simulink model "sm_car"  (R2025a)
settings: Solver=ode23t  StartTime=0.0  StopTime=400  MaxStep=0.4  RelTol=1e-3  AbsTol=1e-3  EnableMultiTasking=on
PreLoadFcn:
  | % Due to usability issue in Repeating Sequence block
  | warning('off','Simulink:Masking:Invalid');
  | 
  | % Eliminate unnecessary warnings in inactive variants
  | % Warnings generated only if you click through inactive variant
  | warning('off','MATLAB:nonExistentField');
  | warning('off','Simulink:Parameters:BlkParamUndefined');
PostLoadFcn:
  | set_param([bdroot '/Vehicle'],'popup_trailer','Off')
  | warning('off','sm:sli:setup:compile:LocalSolverNotSupported')
  | %sm_car_config_maneuver(bdroot,'WOT Braking');
  | sm_car_config_vehicle(bdroot,'false');
  | sm_car_config_logging(bdroot);
InitFcn:
  | sm_car_config_camera;
  | Vehicle = sm_car_vehcfg_checkConfig(Vehicle);
  | sm_car_check_tire_model(bdroot);
StartFcn:
  | tic;
StopFcn:
  | Elapsed_Sim_Time = toc;
  | % disp(['Elapsed Sim Time = ' num2str(Elapsed_Sim_Time)]);
undefined symbols (not defined in the file): Axle1D, AxleIn, Camera, Control, Driver, Free, Init, Maneuver, Pedal, RaceFix, RaceSpin, Scene, ShaftL1, ShaftL2, ShaftR1, ShaftR2, Soft, Stiff, Visual, X, xy_data_car_side, Y, Z
libraries: sm_lib x1546, nesl_utility x528, fl_lib x480, SimscapeFluids_lib x61, sdl_lib x49, simulink x29, ee_lib x7, simulink_extras x6, Linkage_Systems x4, Tire_1x2x x4, AntiRollBar_Systems x2, Linkage_Decoupled x2
(part 60 of 79)

== system sm_car/Vehicle/Vehicle/Chassis/SuspA1/Linkage Decoupled/Steer/Rack Driven Shafts/Driver/Human/Torso ==
  ReferenceFrame : sm_lib/Frames and Transforms/Reference Frame
  Solid : sm_lib/Body Elements/File Solid  ExtGeomFileName=Human_torso.STEP  UnitType=Custom  ExtGeomFileUnits=mm  StepReaderType=HEX  ExportConvexHullGeometry=off  InertiaType=CalculateFromGeometry  BasedOnType=Density  Density=rho_human  DensityUnits=kg/m^3  Mass=0  MassUnits=kg  CenterOfMass=[0 0 0]  CenterOfMassUnits=mm  MomentsOfInertia=[1 1 1]  MomentsOfInertiaUnits=kg*mm^2  ProductsOfInertia=[0 0 0]  ProductsOfInertiaUnits=kg*mm^2  GraphicType=FromGeometry  MarkerShape=Sphere  MarkerSize=10  GraphicVisPropType=SimpleVisualProperties  GraphicDiffuseColor=clr_human  GraphicOpacity=opc_human  GraphicSpecularColor=[0.5 0.5 0.5 1.0]  GraphicAmbientColor=[0.15 0.15 0.15 1.0]  GraphicEmissiveColor=[0.0 0.0 0.0 1.0]  GraphicShininess=75  DoExposeReferenceFrame=on  SerializedFrames=<Frames/>
  Transform : sm_lib/Frames and Transforms/Rigid Transform  RotationMethod=ArbitraryAxis  FollAlignAxisA=+X  BaseAlignAxisA=+Y  FollAlignAxisB=+Y  BaseAlignAxisB=+Z  RotationStandardAxis=+Z  RotationAngle=2.0943951023932  RotationAngleUnits=rad  RotationArbitraryAxis=[-0.577350269189626 -0.577350269189626 0.577350269189626]  RotationSequenceAxes=FollowerAxes  RotationSequence=XYX  RotationSequenceAngles=[0 0 0]  RotationSequenceAnglesUnits=deg  RotationMatrix=[1 0 0; 0 1 0; 0 0 1]  Quaternion=[1 0 0 0]  TranslationMethod=Cartesian  TranslationCartesianOffset=[234.912747775434 20.8274805499988 437.3777771]  TranslationCartesianOffsetUnits=mm  TranslationStandardAxis=+Z  TranslationStandardOffset=0  TranslationStandardOffsetUnits=mm  TranslationROffset=0  TranslationROffsetUnits=m  TranslationThetaOffset=0  TranslationThetaOffsetUnits=deg  TranslationZOffset=0  TranslationZOffsetUnits=m
  Transform Neck : sm_lib/Frames and Transforms/Rigid Transform  RotationMethod=StandardAxis  FollAlignAxisA=+X  BaseAlignAxisA=+Y  FollAlignAxisB=+Y  BaseAlignAxisB=+Z  RotationStandardAxis=+X  RotationAngle=90  RotationAngleUnits=deg  RotationArbitraryAxis=[0 0 1]  RotationSequenceAxes=FollowerAxes  RotationSequence=XYX  RotationSequenceAngles=[0 0 0]  RotationSequenceAnglesUnits=deg  RotationMatrix=[1 0 0; 0 1 0; 0 0 1]  Quaternion=[1 0 0 0]  TranslationMethod=None  TranslationCartesianOffset=[0 0 0]  TranslationCartesianOffsetUnits=m  TranslationStandardAxis=+Z  TranslationStandardOffset=0  TranslationStandardOffsetUnits=m  TranslationROffset=0  TranslationROffsetUnits=m  TranslationThetaOffset=0  TranslationThetaOffsetUnits=deg  TranslationZOffset=0  TranslationZOffsetUnits=m
  Transform Nod : sm_lib/Frames and Transforms/Rigid Transform  RotationMethod=StandardAxis  FollAlignAxisA=+X  BaseAlignAxisA=+Y  FollAlignAxisB=+Y  BaseAlignAxisB=+Z  RotationStandardAxis=+Z  RotationAngle=head_incl_angle  RotationAngleUnits=deg  RotationArbitraryAxis=[0 0 1]  RotationSequenceAxes=FollowerAxes  RotationSequence=XYX  RotationSequenceAngles=[0 0 0]  RotationSequenceAnglesUnits=deg  RotationMatrix=[1 0 0; 0 1 0; 0 0 1]  Quaternion=[1 0 0 0]  TranslationMethod=None  TranslationCartesianOffset=[0 0 0]  TranslationCartesianOffsetUnits=m  TranslationStandardAxis=+Z  TranslationStandardOffset=0  TranslationStandardOffsetUnits=m  TranslationROffset=0  TranslationROffsetUnits=m  TranslationThetaOffset=0  TranslationThetaOffsetUnits=deg  TranslationZOffset=0  TranslationZOffsetUnits=m
  Transform ShoulderL : sm_lib/Frames and Transforms/Rigid Transform  RotationMethod=StandardAxis  FollAlignAxisA=+X  BaseAlignAxisA=+Y  FollAlignAxisB=+Y  BaseAlignAxisB=+Z  RotationStandardAxis=+Y  RotationAngle=90  RotationAngleUnits=deg  RotationArbitraryAxis=[0 0 1]  RotationSequenceAxes=FollowerAxes  RotationSequence=XYX  RotationSequenceAngles=[0 0 0]  RotationSequenceAnglesUnits=deg  RotationMatrix=[1 0 0; 0 1 0; 0 0 1]  Quaternion=[1 0 0 0]  TranslationMethod=StandardAxis  TranslationCartesianOffset=[0 0 0]  TranslationCartesianOffsetUnits=m  TranslationStandardAxis=+Z  TranslationStandardOffset=0.05  TranslationStandardOffsetUnits=m  TranslationROffset=0  TranslationROffsetUnits=m  TranslationThetaOffset=0  TranslationThetaOffsetUnits=deg  TranslationZOffset=0  TranslationZOffsetUnits=m
  Transform ShoulderR : sm_lib/Frames and Transforms/Rigid Transform  RotationMethod=StandardAxis  FollAlignAxisA=+X  BaseAlignAxisA=+Y  FollAlignAxisB=+Y  BaseAlignAxisB=+Z  RotationStandardAxis=+Y  RotationAngle=90  RotationAngleUnits=deg  RotationArbitraryAxis=[0 0 1]  RotationSequenceAxes=FollowerAxes  RotationSequence=XYX  RotationSequenceAngles=[0 0 0]  RotationSequenceAnglesUnits=deg  RotationMatrix=[1 0 0; 0 1 0; 0 0 1]  Quaternion=[1 0 0 0]  TranslationMethod=StandardAxis  TranslationCartesianOffset=[0 0 0]  TranslationCartesianOffsetUnits=m  TranslationStandardAxis=+Z  TranslationStandardOffset=0.05  TranslationStandardOffsetUnits=m  TranslationROffset=0  TranslationROffsetUnits=m  TranslationThetaOffset=0  TranslationThetaOffsetUnits=deg  TranslationZOffset=0  TranslationZOffsetUnits=m
  Transform1 : sm_lib/Frames and Transforms/Rigid Transform  RotationMethod=ArbitraryAxis  FollAlignAxisA=+X  BaseAlignAxisA=+Y  FollAlignAxisB=+Y  BaseAlignAxisB=+Z  RotationStandardAxis=+Z  RotationAngle=2.47638432691423  RotationAngleUnits=rad  RotationArbitraryAxis=[-0.663578618400423 -0.663578618400423 -0.345437164189917]  RotationSequenceAxes=FollowerAxes  RotationSequence=XYX  RotationSequenceAngles=[0 0 0]  RotationSequenceAnglesUnits=deg  RotationMatrix=[1 0 0; 0 1 0; 0 0 1]  Quaternion=[1 0 0 0]  TranslationMethod=Cartesian  TranslationCartesianOffset=[3.33060423509468e-15 -64.9684183409698 16.1065362520158]  TranslationCartesianOffsetUnits=mm  TranslationStandardAxis=+Z  TranslationStandardOffset=0  TranslationStandardOffsetUnits=mm  TranslationROffset=0  TranslationROffsetUnits=m  TranslationThetaOffset=0  TranslationThetaOffsetUnits=deg  TranslationZOffset=0  TranslationZOffsetUnits=m
  Transform2 : sm_lib/Frames and Transforms/Rigid Transform  RotationMethod=ArbitraryAxis  FollAlignAxisA=+X  BaseAlignAxisA=+Y  FollAlignAxisB=+Y  BaseAlignAxisB=+Z  RotationStandardAxis=+Z  RotationAngle=2.0943951023932  RotationAngleUnits=rad  RotationArbitraryAxis=[0.577350269189626 0.577350269189626 0.577350269189626]  RotationSequenceAxes=FollowerAxes  RotationSequence=XYX  RotationSequenceAngles=[0 0 0]  RotationSequenceAnglesUnits=deg  RotationMatrix=[1 0 0; 0 1 0; 0 0 1]  Quaternion=[1 0 0 0]  TranslationMethod=Cartesian  TranslationCartesianOffset=[0 20.82747817 499.8600769]  TranslationCartesianOffsetUnits=mm  TranslationStandardAxis=+Z  TranslationStandardOffset=0  TranslationStandardOffsetUnits=mm  TranslationROffset=0  TranslationROffsetUnits=m  TranslationThetaOffset=0  TranslationThetaOffsetUnits=deg  TranslationZOffset=0  TranslationZOffsetUnits=m
  Transform3 : sm_lib/Frames and Transforms/Rigid Transform  RotationMethod=ArbitraryAxis  FollAlignAxisA=+X  BaseAlignAxisA=+Y  FollAlignAxisB=+Y  BaseAlignAxisB=+Z  RotationStandardAxis=+Z  RotationAngle=2.0943951023932  RotationAngleUnits=rad  RotationArbitraryAxis=[0.577350269189626 0.577350269189626 0.577350269189626]  RotationSequenceAxes=FollowerAxes  RotationSequence=XYX  RotationSequenceAngles=[0 0 0]  RotationSequenceAnglesUnits=deg  RotationMatrix=[1 0 0; 0 1 0; 0 0 1]  Quaternion=[1 0 0 0]  TranslationMethod=Cartesian  TranslationCartesianOffset=[-236.437604017244 20.8274805500079 437.377777100002]  TranslationCartesianOffsetUnits=mm  TranslationStandardAxis=+Z  TranslationStandardOffset=0  TranslationStandardOffsetUnits=mm  TranslationROffset=0  TranslationROffsetUnits=m  TranslationThetaOffset=0  TranslationThetaOffsetUnits=deg  TranslationZOffset=0  TranslationZOffsetUnits=m
  Pelvis : PMIOPort  Side=Left
  ArmL : PMIOPort  Port=2  Side=Right
  Head : PMIOPort  Port=3  Side=Right
  ArmR : PMIOPort  Port=4  Side=Right
  connections:
  Transform Nod/RConn1 -- Transform Neck/LConn1
  Transform/LConn1 -- Transform1/LConn1 -- ReferenceFrame/RConn1 -- Solid/RConn1 -- Transform2/LConn1 -- Transform3/LConn1
  Transform ShoulderL/RConn1 -- ArmL/RConn1
  Transform1/RConn1 -- Pelvis/RConn1
  Transform2/RConn1 -- Transform Nod/LConn1
  Transform3/RConn1 -- Transform ShoulderR/LConn1
  Transform ShoulderR/RConn1 -- ArmR/RConn1
  Transform/RConn1 -- Transform ShoulderL/LConn1
  Transform Neck/RConn1 -- Head/RConn1

== system sm_car/Vehicle/Vehicle/Chassis/SuspA1/Linkage Decoupled/Steer/Rack Driven Shafts/Driver/Human/Twist ==
  Revolute Joint : sm_lib/Joints/Revolute Joint  Commented=on  JointMode=Normal  CompositeWrenchDir=FollowerOnBase  CompositeWrenchFrame=BaseFrame  SenseConstraintForce=off  SenseConstraintTorque=off  SenseTotalForce=off  SenseTotalTorque=off  PositionTargetSpecify=off  PositionTargetPriority=High  PositionTargetValue=0  PositionTargetValueUnits=deg  VelocityTargetSpecify=off  VelocityTargetPriority=High  VelocityTargetValue=0  VelocityTargetValueUnits=deg/s  EquilibriumPosition=0  EquilibriumPositionUnits=deg  SpringStiffness=dt_k  SpringStiffnessUnits=N*m/deg  DampingCoefficient=dt_b  DampingCoefficientUnits=N*m/(deg/s)  LowerLimitSpecify=off  LowerLimitBound=-90  LowerLimitBoundUnits=deg  LowerLimitStiffness=1e4  LowerLimitStiffnessUnits=N*m/deg  LowerLimitDamping=10  LowerLimitDampingUnits=N*m/(deg/s)  LowerLimitTransitionRegionWidth=0.1  LowerLimitTransitionRegionWidthUnits=deg  UpperLimitSpecify=off  UpperLimitBound=90  UpperLimitBoundUnits=deg  UpperLimitStiffness=1e4  UpperLimitStiffnessUnits=N*m/deg  UpperLimitDamping=10  UpperLimitDampingUnits=N*m/(deg/s)  UpperLimitTransitionRegionWidth=0.1  UpperLimitTransitionRegionWidthUnits=deg  TorqueActuationMode=NoTorque  MotionActuationMode=ComputedMotion  SensePosition=off  SenseVelocity=off  SenseAcceleration=off  SenseTorqueForce=off  SenseLowerLimitTorqueForce=off  SenseUpperLimitTorqueForce=off
  Transform Axis Location B : sm_lib/Frames and Transforms/Rigid Transform  RotationMethod=None  FollAlignAxisA=+X  BaseAlignAxisA=+Y  FollAlignAxisB=+Y  BaseAlignAxisB=+Z  RotationStandardAxis=+Y  RotationAngle=0  RotationAngleUnits=deg  RotationArbitraryAxis=[0 0 1]  RotationSequenceAxes=FollowerAxes  RotationSequence=XYX  RotationSequenceAngles=[0 0 0]  RotationSequenceAnglesUnits=deg  RotationMatrix=[1 0 0; 0 1 0; 0 0 1]  Quaternion=[1 0 0 0]  TranslationMethod=StandardAxis  TranslationCartesianOffset=[0 0 0]  TranslationCartesianOffsetUnits=m  TranslationStandardAxis=-X  TranslationStandardOffset=0.05  TranslationStandardOffsetUnits=m  TranslationROffset=0  TranslationROffsetUnits=m  TranslationThetaOffset=0  TranslationThetaOffsetUnits=deg  TranslationZOffset=0  TranslationZOffsetUnits=m
  Transform Axis Location F : sm_lib/Frames and Transforms/Rigid Transform  RotationMethod=None  FollAlignAxisA=+X  BaseAlignAxisA=+Y  FollAlignAxisB=+Y  BaseAlignAxisB=+Z  RotationStandardAxis=+Y  RotationAngle=0  RotationAngleUnits=deg  RotationArbitraryAxis=[0 0 1]  RotationSequenceAxes=FollowerAxes  RotationSequence=XYX  RotationSequenceAngles=[0 0 0]  RotationSequenceAnglesUnits=deg  RotationMatrix=[1 0 0; 0 1 0; 0 0 1]  Quaternion=[1 0 0 0]  TranslationMethod=StandardAxis  TranslationCartesianOffset=[0 0 0]  TranslationCartesianOffsetUnits=m  TranslationStandardAxis=-X  TranslationStandardOffset=0.05  TranslationStandardOffsetUnits=m  TranslationROffset=0  TranslationROffsetUnits=m  TranslationThetaOffset=0  TranslationThetaOffsetUnits=deg  TranslationZOffset=0  TranslationZOffsetUnits=m
  Transform Axis Orientation B : sm_lib/Frames and Transforms/Rigid Transform  RotationMethod=StandardAxis  FollAlignAxisA=+X  BaseAlignAxisA=+Y  FollAlignAxisB=+Y  BaseAlignAxisB=+Z  RotationStandardAxis=+Y  RotationAngle=120  RotationAngleUnits=deg  RotationArbitraryAxis=[0 0 1]  RotationSequenceAxes=FollowerAxes  RotationSequence=XYX  RotationSequenceAngles=[0 0 0]  RotationSequenceAnglesUnits=deg  RotationMatrix=[1 0 0; 0 1 0; 0 0 1]  Quaternion=[1 0 0 0]  TranslationMethod=None  TranslationCartesianOffset=[0 0 0]  TranslationCartesianOffsetUnits=m  TranslationStandardAxis=+Z  TranslationStandardOffset=0  TranslationStandardOffsetUnits=m  TranslationROffset=0  TranslationROffsetUnits=m  TranslationThetaOffset=0  TranslationThetaOffsetUnits=deg  TranslationZOffset=0  TranslationZOffsetUnits=m
  Transform Axis Orientation F : sm_lib/Frames and Transforms/Rigid Transform  RotationMethod=StandardAxis  FollAlignAxisA=+X  BaseAlignAxisA=+Y  FollAlignAxisB=+Y  BaseAlignAxisB=+Z  RotationStandardAxis=+Y  RotationAngle=120  RotationAngleUnits=deg  RotationArbitraryAxis=[0 0 1]  RotationSequenceAxes=FollowerAxes  RotationSequence=XYX  RotationSequenceAngles=[0 0 0]  RotationSequenceAnglesUnits=deg  RotationMatrix=[1 0 0; 0 1 0; 0 0 1]  Quaternion=[1 0 0 0]  TranslationMethod=None  TranslationCartesianOffset=[0 0 0]  TranslationCartesianOffsetUnits=m  TranslationStandardAxis=+Z  TranslationStandardOffset=0  TranslationStandardOffsetUnits=m  TranslationROffset=0  TranslationROffsetUnits=m  TranslationThetaOffset=0  TranslationThetaOffsetUnits=deg  TranslationZOffset=0  TranslationZOffsetUnits=m
  Transform Universal B : sm_lib/Frames and Transforms/Rigid Transform  RotationMethod=StandardAxis  FollAlignAxisA=+X  BaseAlignAxisA=+Y  FollAlignAxisB=+Y  BaseAlignAxisB=+Z  RotationStandardAxis=+Y  RotationAngle=90  RotationAngleUnits=deg  RotationArbitraryAxis=[0 0 1]  RotationSequenceAxes=FollowerAxes  RotationSequence=XYX  RotationSequenceAngles=[0 0 0]  RotationSequenceAnglesUnits=deg  RotationMatrix=[1 0 0; 0 1 0; 0 0 1]  Quaternion=[1 0 0 0]  TranslationMethod=None  TranslationCartesianOffset=[0 0 0]  TranslationCartesianOffsetUnits=m  TranslationStandardAxis=+Z  TranslationStandardOffset=0  TranslationStandardOffsetUnits=m  TranslationROffset=0  TranslationROffsetUnits=m  TranslationThetaOffset=0  TranslationThetaOffsetUnits=deg  TranslationZOffset=0  TranslationZOffsetUnits=m
  Transform Universal F : sm_lib/Frames and Transforms/Rigid Transform  RotationMethod=StandardAxis  FollAlignAxisA=+X  BaseAlignAxisA=+Y  FollAlignAxisB=+Y  BaseAlignAxisB=+Z  RotationStandardAxis=+Y  RotationAngle=90  RotationAngleUnits=deg  RotationArbitraryAxis=[0 0 1]  RotationSequenceAxes=FollowerAxes  RotationSequence=XYX  RotationSequenceAngles=[0 0 0]  RotationSequenceAnglesUnits=deg  RotationMatrix=[1 0 0; 0 1 0; 0 0 1]  Quaternion=[1 0 0 0]  TranslationMethod=None  TranslationCartesianOffset=[0 0 0]  TranslationCartesianOffsetUnits=m  TranslationStandardAxis=+Z  TranslationStandardOffset=0  TranslationStandardOffsetUnits=m  TranslationROffset=0  TranslationROffsetUnits=m  TranslationThetaOffset=0  TranslationThetaOffsetUnits=deg  TranslationZOffset=0  TranslationZOffsetUnits=m
  Universal Torso : sm_lib/Joints/Universal Joint  JointMode=Normal  CompositeWrenchDir=FollowerOnBase  CompositeWrenchFrame=BaseFrame  SenseConstraintForce=off  SenseConstraintTorque=off  SenseTotalForce=off  SenseTotalTorque=off  RxPositionTargetSpecify=off  RxPositionTargetPriority=High  RxPositionTargetValue=0  RxPositionTargetValueUnits=deg  RxVelocityTargetSpecify=off  RxVelocityTargetPriority=High  RxVelocityTargetValue=0  RxVelocityTargetValueUnits=deg/s  RxEquilibriumPosition=0  RxEquilibriumPositionUnits=deg  RxSpringStiffness=10  RxSpringStiffnessUnits=N*m/deg  RxDampingCoefficient=1  RxDampingCoefficientUnits=N*m/(deg/s)  RxLowerLimitSpecify=off  RxLowerLimitBound=-90  RxLowerLimitBoundUnits=deg  RxLowerLimitStiffness=1e4  RxLowerLimitStiffnessUnits=N*m/deg  RxLowerLimitDamping=10  RxLowerLimitDampingUnits=N*m/(deg/s)  RxLowerLimitTransitionRegionWidth=0.1  RxLowerLimitTransitionRegionWidthUnits=deg  RxUpperLimitSpecify=off  RxUpperLimitBound=90  RxUpperLimitBoundUnits=deg  RxUpperLimitStiffness=1e4  RxUpperLimitStiffnessUnits=N*m/deg  RxUpperLimitDamping=10  RxUpperLimitDampingUnits=N*m/(deg/s)  RxUpperLimitTransitionRegionWidth=0.1  RxUpperLimitTransitionRegionWidthUnits=deg  RxTorqueActuationMode=NoTorque  RxMotionActuationMode=ComputedMotion  RxSensePosition=off  RxSenseVelocity=off  RxSenseAcceleration=off  RxSenseTorqueForce=off  RxSenseLowerLimitTorqueForce=off  RxSenseUpperLimitTorqueForce=off  RyPositionTargetSpecify=off  RyPositionTargetPriority=High  RyPositionTargetValue=0  RyPositionTargetValueUnits=deg  RyVelocityTargetSpecify=off  RyVelocityTargetPriority=High  RyVelocityTargetValue=0  RyVelocityTargetValueUnits=deg/s  RyEquilibriumPosition=0  RyEquilibriumPositionUnits=deg  RySpringStiffness=10  RySpringStiffnessUnits=N*m/deg  RyDampingCoefficient=1  RyDampingCoefficientUnits=N*m/(deg/s)  RyLowerLimitSpecify=off  RyLowerLimitBound=-90  RyLowerLimitBoundUnits=deg  RyLowerLimitStiffness=1e4  RyLowerLimitStiffnessUnits=N*m/deg  RyLowerLimitDamping=10  RyLowerLimitDampingUnits=N*m/(deg/s)  RyLowerLimitTransitionRegionWidth=0.1  RyLowerLimitTransitionRegionWidthUnits=deg  RyUpperLimitSpecify=off  RyUpperLimitBound=90  RyUpperLimitBoundUnits=deg  RyUpperLimitStiffness=1e4  RyUpperLimitStiffnessUnits=N*m/deg  RyUpperLimitDamping=10  RyUpperLimitDampingUnits=N*m/(deg/s)  RyUpperLimitTransitionRegionWidth=0.1  RyUpperLimitTransitionRegionWidthUnits=deg  RyTorqueActuationMode=NoTorque  RyMotionActuationMode=ComputedMotion  RySensePosition=off  RySenseVelocity=off  RySenseAcceleration=off  RySenseTorqueForce=off  RySenseLowerLimitTorqueForce=off  RySenseUpperLimitTorqueForce=off
  T : PMIOPort  Side=Right
  B : PMIOPort  Port=2  Side=Left
  connections:
  Universal Torso/RConn1 -- Transform Universal F/RConn1
  Universal Torso/LConn1 -- Transform Universal B/RConn1
  Transform Axis Location F/RConn1 -- Transform Universal F/LConn1
  Transform Axis Orientation F/LConn1 -- T/RConn1
  Transform Axis Location B/RConn1 -- Transform Universal B/LConn1
  Transform Axis Orientation F/RConn1 -- Transform Axis Location F/LConn1
  B/RConn1 -- Transform Axis Orientation B/LConn1
  Transform Axis Orientation B/RConn1 -- Transform Axis Location B/LConn1

== system sm_car/Vehicle/Vehicle/Chassis/SuspA1/Linkage Decoupled/Steer/Rack Driven Shafts/Driver/None/Body Sensor Empty ==
  Constant{,1..14} (15 alike) : Constant  Value=0
  Reference Frame : sm_lib/Frames and Transforms/Reference Frame
  Signal Specification : SignalSpecification  Unit=rad
  Signal Specification1 : SignalSpecification  Unit=rad
  Signal Specification2 : SignalSpecification  Unit=rad
  Signal Specification3 : SignalSpecification  Unit=rad/s
  Signal Specification4 : SignalSpecification  Unit=rad/s
  Signal Specification5 : SignalSpecification  Unit=rad/s
  B : PMIOPort  Side=Left
  Bus Element Out : Outport  VectorParamsAs1DForOutWhenUnconnected=off  PortName=Body  Element=x
  Bus Element Out1 : Outport  VectorParamsAs1DForOutWhenUnconnected=off  PortName=Body  Element=y
  Bus Element Out2 : Outport  VectorParamsAs1DForOutWhenUnconnected=off  PortName=Body  Element=z
  Bus Element Out3 : Outport  VectorParamsAs1DForOutWhenUnconnected=off  PortName=Body  Element=vx
  Bus Element Out4 : Outport  VectorParamsAs1DForOutWhenUnconnected=off  PortName=Body  Element=vy
  Bus Element Out5 : Outport  VectorParamsAs1DForOutWhenUnconnected=off  PortName=Body  Element=vz
  Bus Element Out6 : Outport  VectorParamsAs1DForOutWhenUnconnected=off  PortName=Body  Element=gx
  Bus Element Out7 : Outport  VectorParamsAs1DForOutWhenUnconnected=off  PortName=Body  Element=gy
  Bus Element Out8 : Outport  VectorParamsAs1DForOutWhenUnconnected=off  PortName=Body  Element=gz
  Bus Element Out9 : Outport  VectorParamsAs1DForOutWhenUnconnected=off  PortName=Body  Element=nRoll
  Bus Element Out10 : Outport  VectorParamsAs1DForOutWhenUnconnected=off  PortName=Body  Element=nPitch
  Bus Element Out11 : Outport  VectorParamsAs1DForOutWhenUnconnected=off  PortName=Body  Element=nYaw
  Bus Element Out12 : Outport  VectorParamsAs1DForOutWhenUnconnected=off  PortName=Body  Element=aRoll
  Bus Element Out13 : Outport  VectorParamsAs1DForOutWhenUnconnected=off  PortName=Body  Element=aPitch
  Bus Element Out14 : Outport  VectorParamsAs1DForOutWhenUnconnected=off  PortName=Body  Element=aYaw
  wires:
  Constant2/1 -> Signal Specification/1
  Constant3/1 -> Signal Specification1/1
  Constant5/1 -> Signal Specification4/1
  Constant4/1 -> Signal Specification3/1
  Constant1/1 -> Signal Specification5/1
  Constant/1 -> Signal Specification2/1
  Signal Specification5/1 -> Bus Element Out11/1
  Signal Specification4/1 -> Bus Element Out10/1
  Signal Specification3/1 -> Bus Element Out9/1
  Signal Specification2/1 -> Bus Element Out14/1
  Signal Specification1/1 -> Bus Element Out13/1
  Signal Specification/1 -> Bus Element Out12/1
  Constant9/1 -> Bus Element Out3/1
  Constant6/1 -> Bus Element Out/1
  Constant8/1 -> Bus Element Out2/1
  Constant10/1 -> Bus Element Out4/1
  Constant13/1 -> Bus Element Out7/1
  Constant7/1 -> Bus Element Out1/1
  Constant12/1 -> Bus Element Out6/1
  Constant11/1 -> Bus Element Out5/1
  Constant14/1 -> Bus Element Out8/1
  connections:
  B/RConn1 -- Reference Frame/RConn1

== system sm_car/Vehicle/Vehicle/Chassis/SuspA1/Linkage Decoupled/Steer/Rack Driven Shafts/Wheel/FSAE/Transform Steer Axis ==
  Rigid Transform1 : sm_lib/Frames and Transforms/Rigid Transform  RotationMethod=None  FollAlignAxisA=+X  BaseAlignAxisA=+Y  FollAlignAxisB=+Y  BaseAlignAxisB=+Z  RotationStandardAxis=+Z  RotationAngle=0.0  RotationAngleUnits=deg  RotationArbitraryAxis=[0 0 1]  RotationSequenceAxes=FollowerAxes  RotationSequence=XYX  RotationSequenceAngles=[0 0 0]  RotationSequenceAnglesUnits=deg  RotationMatrix=[1 0 0; 0 1 0; 0 0 1]  Quaternion=[1 0 0 0]  TranslationMethod=Cartesian  TranslationCartesianOffset=[0 -0.4664 -0.3791]  TranslationCartesianOffsetUnits=m  TranslationStandardAxis=+Z  TranslationStandardOffset=0  TranslationStandardOffsetUnits=m  TranslationROffset=0  TranslationROffsetUnits=m  TranslationThetaOffset=0  TranslationThetaOffsetUnits=deg  TranslationZOffset=0  TranslationZOffsetUnits=m
  Rigid Transform2 : sm_lib/Frames and Transforms/Rigid Transform  RotationMethod=RotationMatrix  FollAlignAxisA=+X  BaseAlignAxisA=+Y  FollAlignAxisB=+Y  BaseAlignAxisB=+Z  RotationStandardAxis=+Z  RotationAngle=0.0  RotationAngleUnits=deg  RotationArbitraryAxis=[0 0 1]  RotationSequenceAxes=FollowerAxes  RotationSequence=XYX  RotationSequenceAngles=[0 0 0]  RotationSequenceAnglesUnits=deg  RotationMatrix=[0.5 0.866 -6.661e-16; -0.8602 0.4967 0.1153; 0.09988 -0.05766 0.9933]  Quaternion=[1 0 0 0]  TranslationMethod=None  TranslationCartesianOffset=[0 0 0]  TranslationCartesianOffsetUnits=m  TranslationStandardAxis=+Z  TranslationStandardOffset=0  TranslationStandardOffsetUnits=m  TranslationROffset=0  TranslationROffsetUnits=m  TranslationThetaOffset=0  TranslationThetaOffsetUnits=deg  TranslationZOffset=0  TranslationZOffsetUnits=m
  Rigid Transform4 : sm_lib/Frames and Transforms/Rigid Transform  RotationMethod=StandardAxis  FollAlignAxisA=+X  BaseAlignAxisA=+Y  FollAlignAxisB=+Y  BaseAlignAxisB=+Z  RotationStandardAxis=+Z  RotationAngle=150  RotationAngleUnits=deg  RotationArbitraryAxis=[0 0 1]  RotationSequenceAxes=FollowerAxes  RotationSequence=XYX  RotationSequenceAngles=[0 0 0]  RotationSequenceAnglesUnits=deg  RotationMatrix=[1 0 0; 0 1 0; 0 0 1]  Quaternion=[1 0 0 0]  TranslationMethod=StandardAxis  TranslationCartesianOffset=[0 0 0]  TranslationCartesianOffsetUnits=m  TranslationStandardAxis=+Z  TranslationStandardOffset=0.09  TranslationStandardOffsetUnits=m  TranslationROffset=0  TranslationROffsetUnits=m  TranslationThetaOffset=0  TranslationThetaOffsetUnits=deg  TranslationZOffset=0  TranslationZOffsetUnits=m
  F : PMIOPort  Side=Left
  B : PMIOPort  Port=2  Side=Right
  connections:
  B/RConn1 -- Rigid Transform1/RConn1
  Rigid Transform1/LConn1 -- Rigid Transform2/LConn1
  F/RConn1 -- Rigid Transform4/RConn1
  Rigid Transform2/RConn1 -- Rigid Transform4/LConn1

== system sm_car/Vehicle/Vehicle/Chassis/SuspA1/Linkage Decoupled/Steer/Rack Driven Shafts/Wheel/Sedan/Steering ==
  Steering Wheel : sm_lib/Body Elements/File Solid  ExtGeomFileName=Sedan_Hamba_Steering_Wheel.stl  UnitType=Custom  ExtGeomFileUnits=m  StepReaderType=HEX  ExportConvexHullGeometry=off  InertiaType=CalculateFromGeometry  BasedOnType=Density  Density=1000  DensityUnits=kg/m^3  Mass=0  MassUnits=kg  CenterOfMass=[0 0 0]  CenterOfMassUnits=m  MomentsOfInertia=[1 1 1]  MomentsOfInertiaUnits=kg*m^2  ProductsOfInertia=[0 0 0]  ProductsOfInertiaUnits=kg*m^2  GraphicType=FromGeometry  MarkerShape=Sphere  MarkerSize=10  GraphicVisPropType=SimpleVisualProperties  GraphicDiffuseColor=[0.4 0.4 0.4]  GraphicOpacity=1.0  GraphicSpecularColor=[0.5 0.5 0.5 1.0]  GraphicAmbientColor=[0.15 0.15 0.15 1.0]  GraphicEmissiveColor=[0.0 0.0 0.0 1.0]  GraphicShininess=75  DoExposeReferenceFrame=on  SerializedFrames=<Frames/>
  Transform Bot Ctr : sm_lib/Frames and Transforms/Rigid Transform  RotationMethod=None  FollAlignAxisA=+X  BaseAlignAxisA=+Y  FollAlignAxisB=+Y  BaseAlignAxisB=+Z  RotationStandardAxis=+Z  RotationAngle=0.0  RotationAngleUnits=deg  RotationArbitraryAxis=[0 0 1]  RotationSequenceAxes=FollowerAxes  RotationSequence=XYX  RotationSequenceAngles=[0 0 0]  RotationSequenceAnglesUnits=deg  RotationMatrix=[1 0 0; 0 1 0; 0 0 1]  Quaternion=[1 0 0 0]  TranslationMethod=Cartesian  TranslationCartesianOffset="[-0.020653016865253  -0.076110564172268   0.210841685533524]"  TranslationCartesianOffsetUnits=m  TranslationStandardAxis=+Z  TranslationStandardOffset=0  TranslationStandardOffsetUnits=m  TranslationROffset=0  TranslationROffsetUnits=m  TranslationThetaOffset=0  TranslationThetaOffsetUnits=deg  TranslationZOffset=0  TranslationZOffsetUnits=m
  Transform Location : sm_lib/Frames and Transforms/Rigid Transform  RotationMethod=None  FollAlignAxisA=+X  BaseAlignAxisA=+Y  FollAlignAxisB=+Y  BaseAlignAxisB=+Z  RotationStandardAxis=+Z  RotationAngle=0.0  RotationAngleUnits=deg  RotationArbitraryAxis=[0 0 1]  RotationSequenceAxes=FollowerAxes  RotationSequence=XYX  RotationSequenceAngles=[0 0 0]  RotationSequenceAnglesUnits=deg  RotationMatrix=[1 0 0; 0 1 0; 0 0 1]  Quaternion=[1 0 0 0]  TranslationMethod=Cartesian  TranslationCartesianOffset=[0.5868 -0.3915 -0.838]  TranslationCartesianOffsetUnits=m  TranslationStandardAxis=+Z  TranslationStandardOffset=0  TranslationStandardOffsetUnits=m  TranslationROffset=0  TranslationROffsetUnits=m  TranslationThetaOffset=0  TranslationThetaOffsetUnits=deg  TranslationZOffset=0  TranslationZOffsetUnits=m
  Transform Orientation : sm_lib/Frames and Transforms/Rigid Transform  RotationMethod=RotationSequence  FollAlignAxisA=+X  BaseAlignAxisA=+Y  FollAlignAxisB=+Y  BaseAlignAxisB=+Z  RotationStandardAxis=+Z  RotationAngle=0.0  RotationAngleUnits=deg  RotationArbitraryAxis=[0 0 1]  RotationSequenceAxes=FollowerAxes  RotationSequence=ZYX  RotationSequenceAngles=[-90 -90 0]  RotationSequenceAnglesUnits=deg  RotationMatrix=[1 0 0; 0 1 0; 0 0 1]  Quaternion=[1 0 0 0]  TranslationMethod=None  TranslationCartesianOffset=[0 0 0]  TranslationCartesianOffsetUnits=m  TranslationStandardAxis=+Z  TranslationStandardOffset=0  TranslationStandardOffsetUnits=m  TranslationROffset=0  TranslationROffsetUnits=m  TranslationThetaOffset=0  TranslationThetaOffsetUnits=deg  TranslationZOffset=0  TranslationZOffsetUnits=m
  Transform Top Ctr : sm_lib/Frames and Transforms/Rigid Transform  RotationMethod=None  FollAlignAxisA=+X  BaseAlignAxisA=+Y  FollAlignAxisB=+Y  BaseAlignAxisB=+Z  RotationStandardAxis=+Z  RotationAngle=0.0  RotationAngleUnits=deg  RotationArbitraryAxis=[0 0 1]  RotationSequenceAxes=FollowerAxes  RotationSequence=XYX  RotationSequenceAngles=[0 0 0]  RotationSequenceAnglesUnits=deg  RotationMatrix=[1 0 0; 0 1 0; 0 0 1]  Quaternion=[1 0 0 0]  TranslationMethod=Cartesian  TranslationCartesianOffset="[0.124706447124481   0.318579733371735   0.210841685533524]"  TranslationCartesianOffsetUnits=m  TranslationStandardAxis=+Z  TranslationStandardOffset=0  TranslationStandardOffsetUnits=m  TranslationROffset=0  TranslationROffsetUnits=m  TranslationThetaOffset=0  TranslationThetaOffsetUnits=deg  TranslationZOffset=0  TranslationZOffsetUnits=m
  R : PMIOPort  Side=Right
  BotCtr : PMIOPort  Port=2  Side=Left
  TopCtr : PMIOPort  Port=3  Side=Left
  connections:
  Transform Bot Ctr/LConn1 -- Transform Orientation/LConn1 -- R/RConn1 -- Transform Top Ctr/LConn1
  Transform Location/RConn1 -- Steering Wheel/RConn1
  Transform Orientation/RConn1 -- Transform Location/LConn1
  Transform Bot Ctr/RConn1 -- BotCtr/RConn1
  TopCtr/RConn1 -- Transform Top Ctr/RConn1

== system sm_car/Vehicle/Vehicle/Chassis/SuspA1/Linkage Decoupled/Steer/Rack Static Shafts/Driver/Human/Arm L ==
  Arm Lower L : Subsystem
  Arm Upper L : Subsystem
  Hand L : Subsystem
  Revolute ElbowL : sm_lib/Joints/Revolute Joint  JointMode=Normal  CompositeWrenchDir=FollowerOnBase  CompositeWrenchFrame=BaseFrame  SenseConstraintForce=off  SenseConstraintTorque=off  SenseTotalForce=off  SenseTotalTorque=off  PositionTargetSpecify=on  PositionTargetPriority=Low  PositionTargetValue=50  PositionTargetValueUnits=deg  VelocityTargetSpecify=off  VelocityTargetPriority=High  VelocityTargetValue=0  VelocityTargetValueUnits=deg/s  EquilibriumPosition=0  EquilibriumPositionUnits=deg  SpringStiffness=0  SpringStiffnessUnits=N*m/deg  DampingCoefficient=0  DampingCoefficientUnits=N*m/(deg/s)  LowerLimitSpecify=off  LowerLimitBound=-90  LowerLimitBoundUnits=deg  LowerLimitStiffness=1e4  LowerLimitStiffnessUnits=N*m/deg  LowerLimitDamping=10  LowerLimitDampingUnits=N*m/(deg/s)  LowerLimitTransitionRegionWidth=0.1  LowerLimitTransitionRegionWidthUnits=deg  UpperLimitSpecify=off  UpperLimitBound=90  UpperLimitBoundUnits=deg  UpperLimitStiffness=1e4  UpperLimitStiffnessUnits=N*m/deg  UpperLimitDamping=10  UpperLimitDampingUnits=N*m/(deg/s)  UpperLimitTransitionRegionWidth=0.1  UpperLimitTransitionRegionWidthUnits=deg  TorqueActuationMode=NoTorque  MotionActuationMode=ComputedMotion  SensePosition=off  SenseVelocity=off  SenseAcceleration=off  SenseTorqueForce=off  SenseLowerLimitTorqueForce=off  SenseUpperLimitTorqueForce=off
  Spherical ShoulderL : sm_lib/Joints/Spherical Joint  JointMode=Normal  CompositeWrenchDir=FollowerOnBase  CompositeWrenchFrame=BaseFrame  SenseConstraintForce=off  SenseConstraintTorque=off  SenseTotalForce=off  SenseTotalTorque=off  PositionTargetSpecify=off  PositionTargetPriority=High  PositionTargetRotationMethod=None  PositionTargetFollAlignAxisA=+X  PositionTargetBaseAlignAxisA=+Y  PositionTargetFollAlignAxisB=+Y  PositionTargetBaseAlignAxisB=+Z  PositionTargetRotationStandardAxis=+Z  PositionTargetRotationAngle=0.0  PositionTargetRotationAngleUnits=deg  PositionTargetRotationArbitraryAxis=[0 0 1]  PositionTargetRotationSequenceAxes=FollowerAxes  PositionTargetRotationSequence=XYX  PositionTargetRotationSequenceAngles=[0 0 0]  PositionTargetRotationSequenceAnglesUnits=deg  PositionTargetRotationMatrix=[1 0 0; 0 1 0; 0 0 1]  PositionTargetQuaternion=[1 0 0 0]  VelocityTargetSpecify=off  VelocityTargetPriority=High  VelocityTargetValue=[0 0 0]  VelocityTargetValueUnits=deg/s  VelocityTargetInFollowerFrame=on  EqPosRotationMethod=None  EqPosFollAlignAxisA=+X  EqPosBaseAlignAxisA=+Y  EqPosFollAlignAxisB=+Y  EqPosBaseAlignAxisB=+Z  EqPosRotationStandardAxis=+Z  EqPosRotationAngle=0.0  EqPosRotationAngleUnits=deg  EqPosRotationArbitraryAxis=[0 0 1]  EqPosRotationSequenceAxes=FollowerAxes  EqPosRotationSequence=XYX  EqPosRotationSequenceAngles=[0 0 0]  EqPosRotationSequenceAnglesUnits=deg  EqPosRotationMatrix=[1 0 0; 0 1 0; 0 0 1]  EqPosQuaternion=[1 0 0 0]  SpringStiffness=0  SpringStiffnessUnits=N*m/deg  DampingCoefficient=0  DampingCoefficientUnits=N*m/(deg/s)  LowerLimitSpecify=off  LowerLimitBound=15  LowerLimitBoundUnits=deg  LowerLimitStiffness=1e4  LowerLimitStiffnessUnits=N*m/deg  LowerLimitDamping=10  LowerLimitDampingUnits=N*m/(deg/s)  LowerLimitTransitionRegionWidth=0.1  LowerLimitTransitionRegionWidthUnits=deg  UpperLimitSpecify=off  UpperLimitBound=45  UpperLimitBoundUnits=deg  UpperLimitStiffness=1e4  UpperLimitStiffnessUnits=N*m/deg  UpperLimitDamping=10  UpperLimitDampingUnits=N*m/(deg/s)  UpperLimitTransitionRegionWidth=0.1  UpperLimitTransitionRegionWidthUnits=deg  TorqueActuationMode=NoTorque  ActuateTorqueX=off  ActuateTorqueY=off  ActuateTorqueZ=off  ActuateTorque=off  ActuationFrame=BaseFrame  SensePosition=off  SenseVelocityX=off  SenseVelocityY=off  SenseVelocityZ=off  SenseVelocity=off  SenseAccelerationX=off  SenseAccelerationY=off  SenseAccelerationZ=off  SenseAcceleration=off  SenseLowerLimitTorqueMag=off  SenseUpperLimitTorqueMag=off  SensingFrame=BaseFrame
  Universal WristL : sm_lib/Joints/Universal Joint  JointMode=Normal  CompositeWrenchDir=FollowerOnBase  CompositeWrenchFrame=BaseFrame  SenseConstraintForce=off  SenseConstraintTorque=off  SenseTotalForce=off  SenseTotalTorque=off  RxPositionTargetSpecify=off  RxPositionTargetPriority=High  RxPositionTargetValue=0  RxPositionTargetValueUnits=deg  RxVelocityTargetSpecify=off  RxVelocityTargetPriority=High  RxVelocityTargetValue=0  RxVelocityTargetValueUnits=deg/s  RxEquilibriumPosition=0  RxEquilibriumPositionUnits=deg  RxSpringStiffness=0  RxSpringStiffnessUnits=N*m/deg  RxDampingCoefficient=0  RxDampingCoefficientUnits=N*m/(deg/s)  RxLowerLimitSpecify=off  RxLowerLimitBound=-90  RxLowerLimitBoundUnits=deg  RxLowerLimitStiffness=1e4  RxLowerLimitStiffnessUnits=N*m/deg  RxLowerLimitDamping=10  RxLowerLimitDampingUnits=N*m/(deg/s)  RxLowerLimitTransitionRegionWidth=0.1  RxLowerLimitTransitionRegionWidthUnits=deg  RxUpperLimitSpecify=off  RxUpperLimitBound=90  RxUpperLimitBoundUnits=deg  RxUpperLimitStiffness=1e4  RxUpperLimitStiffnessUnits=N*m/deg  RxUpperLimitDamping=10  RxUpperLimitDampingUnits=N*m/(deg/s)  RxUpperLimitTransitionRegionWidth=0.1  RxUpperLimitTransitionRegionWidthUnits=deg  RxTorqueActuationMode=NoTorque  RxMotionActuationMode=ComputedMotion  RxSensePosition=off  RxSenseVelocity=off  RxSenseAcceleration=off  RxSenseTorqueForce=off  RxSenseLowerLimitTorqueForce=off  RxSenseUpperLimitTorqueForce=off  RyPositionTargetSpecify=off  RyPositionTargetPriority=High  RyPositionTargetValue=0  RyPositionTargetValueUnits=deg  RyVelocityTargetSpecify=off  RyVelocityTargetPriority=High  RyVelocityTargetValue=0  RyVelocityTargetValueUnits=deg/s  RyEquilibriumPosition=0  RyEquilibriumPositionUnits=deg  RySpringStiffness=0  RySpringStiffnessUnits=N*m/deg  RyDampingCoefficient=0  RyDampingCoefficientUnits=N*m/(deg/s)  RyLowerLimitSpecify=off  RyLowerLimitBound=-90  RyLowerLimitBoundUnits=deg  RyLowerLimitStiffness=1e4  RyLowerLimitStiffnessUnits=N*m/deg  RyLowerLimitDamping=10  RyLowerLimitDampingUnits=N*m/(deg/s)  RyLowerLimitTransitionRegionWidth=0.1  RyLowerLimitTransitionRegionWidthUnits=deg  RyUpperLimitSpecify=off  RyUpperLimitBound=90  RyUpperLimitBoundUnits=deg  RyUpperLimitStiffness=1e4  RyUpperLimitStiffnessUnits=N*m/deg  RyUpperLimitDamping=10  RyUpperLimitDampingUnits=N*m/(deg/s)  RyUpperLimitTransitionRegionWidth=0.1  RyUpperLimitTransitionRegionWidthUnits=deg  RyTorqueActuationMode=NoTorque  RyMotionActuationMode=ComputedMotion  RySensePosition=off  RySenseVelocity=off  RySenseAcceleration=off  RySenseTorqueForce=off  RySenseLowerLimitTorqueForce=off  RySenseUpperLimitTorqueForce=off
  Sh : PMIOPort  Side=Left
  Grip : PMIOPort  Port=2  Side=Right
  connections:
  Revolute ElbowL/LConn1 -- Arm Upper L/RConn1
  Spherical ShoulderL/RConn1 -- Arm Upper L/LConn1
  Universal WristL/RConn1 -- Hand L/LConn1
  Hand L/RConn1 -- Grip/RConn1
  Arm Lower L/LConn1 -- Revolute ElbowL/RConn1
  Arm Lower L/RConn1 -- Universal WristL/LConn1
  Spherical ShoulderL/LConn1 -- Sh/RConn1

== system sm_car/Vehicle/Vehicle/Chassis/SuspA1/Linkage Decoupled/Steer/Rack Static Shafts/Driver/Human/Arm R ==
  Arm Lower R : Subsystem
  Arm Upper R : Subsystem
  Hand R : Subsystem
  Revolute ElbowR : sm_lib/Joints/Revolute Joint  JointMode=Normal  CompositeWrenchDir=FollowerOnBase  CompositeWrenchFrame=BaseFrame  SenseConstraintForce=off  SenseConstraintTorque=off  SenseTotalForce=off  SenseTotalTorque=off  PositionTargetSpecify=on  PositionTargetPriority=Low  PositionTargetValue=50  PositionTargetValueUnits=deg  VelocityTargetSpecify=off  VelocityTargetPriority=High  VelocityTargetValue=0  VelocityTargetValueUnits=deg/s  EquilibriumPosition=0  EquilibriumPositionUnits=deg  SpringStiffness=0  SpringStiffnessUnits=N*m/deg  DampingCoefficient=0  DampingCoefficientUnits=N*m/(deg/s)  LowerLimitSpecify=off  LowerLimitBound=-90  LowerLimitBoundUnits=deg  LowerLimitStiffness=1e4  LowerLimitStiffnessUnits=N*m/deg  LowerLimitDamping=10  LowerLimitDampingUnits=N*m/(deg/s)  LowerLimitTransitionRegionWidth=0.1  LowerLimitTransitionRegionWidthUnits=deg  UpperLimitSpecify=off  UpperLimitBound=90  UpperLimitBoundUnits=deg  UpperLimitStiffness=1e4  UpperLimitStiffnessUnits=N*m/deg  UpperLimitDamping=10  UpperLimitDampingUnits=N*m/(deg/s)  UpperLimitTransitionRegionWidth=0.1  UpperLimitTransitionRegionWidthUnits=deg  TorqueActuationMode=NoTorque  MotionActuationMode=ComputedMotion  SensePosition=off  SenseVelocity=off  SenseAcceleration=off  SenseTorqueForce=off  SenseLowerLimitTorqueForce=off  SenseUpperLimitTorqueForce=off
  Spherical ShoulderR : sm_lib/Joints/Spherical Joint  JointMode=Normal  CompositeWrenchDir=FollowerOnBase  CompositeWrenchFrame=BaseFrame  SenseConstraintForce=off  SenseConstraintTorque=off  SenseTotalForce=off  SenseTotalTorque=off  PositionTargetSpecify=off  PositionTargetPriority=High  PositionTargetRotationMethod=None  PositionTargetFollAlignAxisA=+X  PositionTargetBaseAlignAxisA=+Y  PositionTargetFollAlignAxisB=+Y  PositionTargetBaseAlignAxisB=+Z  PositionTargetRotationStandardAxis=+Z  PositionTargetRotationAngle=0.0  PositionTargetRotationAngleUnits=deg  PositionTargetRotationArbitraryAxis=[0 0 1]  PositionTargetRotationSequenceAxes=FollowerAxes  PositionTargetRotationSequence=XYX  PositionTargetRotationSequenceAngles=[0 0 0]  PositionTargetRotationSequenceAnglesUnits=deg  PositionTargetRotationMatrix=[1 0 0; 0 1 0; 0 0 1]  PositionTargetQuaternion=[1 0 0 0]  VelocityTargetSpecify=off  VelocityTargetPriority=High  VelocityTargetValue=[0 0 0]  VelocityTargetValueUnits=deg/s  VelocityTargetInFollowerFrame=on  EqPosRotationMethod=None  EqPosFollAlignAxisA=+X  EqPosBaseAlignAxisA=+Y  EqPosFollAlignAxisB=+Y  EqPosBaseAlignAxisB=+Z  EqPosRotationStandardAxis=+Z  EqPosRotationAngle=0.0  EqPosRotationAngleUnits=deg  EqPosRotationArbitraryAxis=[0 0 1]  EqPosRotationSequenceAxes=FollowerAxes  EqPosRotationSequence=XYX  EqPosRotationSequenceAngles=[0 0 0]  EqPosRotationSequenceAnglesUnits=deg  EqPosRotationMatrix=[1 0 0; 0 1 0; 0 0 1]  EqPosQuaternion=[1 0 0 0]  SpringStiffness=0  SpringStiffnessUnits=N*m/deg  DampingCoefficient=0  DampingCoefficientUnits=N*m/(deg/s)  LowerLimitSpecify=off  LowerLimitBound=15  LowerLimitBoundUnits=deg  LowerLimitStiffness=1e4  LowerLimitStiffnessUnits=N*m/deg  LowerLimitDamping=10  LowerLimitDampingUnits=N*m/(deg/s)  LowerLimitTransitionRegionWidth=0.1  LowerLimitTransitionRegionWidthUnits=deg  UpperLimitSpecify=off  UpperLimitBound=45  UpperLimitBoundUnits=deg  UpperLimitStiffness=1e4  UpperLimitStiffnessUnits=N*m/deg  UpperLimitDamping=10  UpperLimitDampingUnits=N*m/(deg/s)  UpperLimitTransitionRegionWidth=0.1  UpperLimitTransitionRegionWidthUnits=deg  TorqueActuationMode=NoTorque  ActuateTorqueX=off  ActuateTorqueY=off  ActuateTorqueZ=off  ActuateTorque=off  ActuationFrame=BaseFrame  SensePosition=off  SenseVelocityX=off  SenseVelocityY=off  SenseVelocityZ=off  SenseVelocity=off  SenseAccelerationX=off  SenseAccelerationY=off  SenseAccelerationZ=off  SenseAcceleration=off  SenseLowerLimitTorqueMag=off  SenseUpperLimitTorqueMag=off  SensingFrame=BaseFrame
  Universal WristR : sm_lib/Joints/Universal Joint  JointMode=Normal  CompositeWrenchDir=FollowerOnBase  CompositeWrenchFrame=BaseFrame  SenseConstraintForce=off  SenseConstraintTorque=off  SenseTotalForce=off  SenseTotalTorque=off  RxPositionTargetSpecify=off  RxPositionTargetPriority=High  RxPositionTargetValue=0  RxPositionTargetValueUnits=deg  RxVelocityTargetSpecify=off  RxVelocityTargetPriority=High  RxVelocityTargetValue=0  RxVelocityTargetValueUnits=deg/s  RxEquilibriumPosition=0  RxEquilibriumPositionUnits=deg  RxSpringStiffness=0  RxSpringStiffnessUnits=N*m/deg  RxDampingCoefficient=0  RxDampingCoefficientUnits=N*m/(deg/s)  RxLowerLimitSpecify=off  RxLowerLimitBound=-90  RxLowerLimitBoundUnits=deg  RxLowerLimitStiffness=1e4  RxLowerLimitStiffnessUnits=N*m/deg  RxLowerLimitDamping=10  RxLowerLimitDampingUnits=N*m/(deg/s)  RxLowerLimitTransitionRegionWidth=0.1  RxLowerLimitTransitionRegionWidthUnits=deg  RxUpperLimitSpecify=off  RxUpperLimitBound=90  RxUpperLimitBoundUnits=deg  RxUpperLimitStiffness=1e4  RxUpperLimitStiffnessUnits=N*m/deg  RxUpperLimitDamping=10  RxUpperLimitDampingUnits=N*m/(deg/s)  RxUpperLimitTransitionRegionWidth=0.1  RxUpperLimitTransitionRegionWidthUnits=deg  RxTorqueActuationMode=NoTorque  RxMotionActuationMode=ComputedMotion  RxSensePosition=off  RxSenseVelocity=off  RxSenseAcceleration=off  RxSenseTorqueForce=off  RxSenseLowerLimitTorqueForce=off  RxSenseUpperLimitTorqueForce=off  RyPositionTargetSpecify=off  RyPositionTargetPriority=High  RyPositionTargetValue=0  RyPositionTargetValueUnits=deg  RyVelocityTargetSpecify=off  RyVelocityTargetPriority=High  RyVelocityTargetValue=0  RyVelocityTargetValueUnits=deg/s  RyEquilibriumPosition=0  RyEquilibriumPositionUnits=deg  RySpringStiffness=0  RySpringStiffnessUnits=N*m/deg  RyDampingCoefficient=0  RyDampingCoefficientUnits=N*m/(deg/s)  RyLowerLimitSpecify=off  RyLowerLimitBound=-90  RyLowerLimitBoundUnits=deg  RyLowerLimitStiffness=1e4  RyLowerLimitStiffnessUnits=N*m/deg  RyLowerLimitDamping=10  RyLowerLimitDampingUnits=N*m/(deg/s)  RyLowerLimitTransitionRegionWidth=0.1  RyLowerLimitTransitionRegionWidthUnits=deg  RyUpperLimitSpecify=off  RyUpperLimitBound=90  RyUpperLimitBoundUnits=deg  RyUpperLimitStiffness=1e4  RyUpperLimitStiffnessUnits=N*m/deg  RyUpperLimitDamping=10  RyUpperLimitDampingUnits=N*m/(deg/s)  RyUpperLimitTransitionRegionWidth=0.1  RyUpperLimitTransitionRegionWidthUnits=deg  RyTorqueActuationMode=NoTorque  RyMotionActuationMode=ComputedMotion  RySensePosition=off  RySenseVelocity=off  RySenseAcceleration=off  RySenseTorqueForce=off  RySenseLowerLimitTorqueForce=off  RySenseUpperLimitTorqueForce=off
  Grip : PMIOPort  Side=Right
  Sh : PMIOPort  Port=2  Side=Left
  connections:
  Sh/RConn1 -- Spherical ShoulderR/LConn1
  Arm Lower R/RConn1 -- Universal WristR/LConn1
  Arm Upper R/LConn1 -- Spherical ShoulderR/RConn1
  Universal WristR/RConn1 -- Hand R/LConn1
  Revolute ElbowR/RConn1 -- Arm Lower R/LConn1
  Arm Upper R/RConn1 -- Revolute ElbowR/LConn1
  Hand R/RConn1 -- Grip/RConn1
